simulink model "LunarMicrogrid_Full"  (R2026b)
settings: Solver=ode23t  StopTime=simulation.timeSim  MaxStep=1/(5*solarPlant.converterSwitchingFrequency)  AbsTol=1e-3
PreLoadFcn:
  | run('LunarMicrogridA_Data');
values from neighbouring files (symbols this model uses):
  Csc = Csc_cell/Ns_sc*Np_sc    (= 200)    [LunarDAB_Params.m]
  eta_sc = 0.95    [LunarDAB_Params.m]
  fsw = 100e3    (= 100000)    [LunarDAB_Params.m]
  k_restore = 1    [LunarDAB_Params.m]
  kiCurrent = 2    [LunarDAB_Params.m]
  kiVoltage = 8    [LunarDAB_Params.m]
  kpCurrent = 0.005    [LunarDAB_Params.m]
  kpVoltage = 0.4    [LunarDAB_Params.m]
  lTotal = lSeries + Llk    [LunarDAB_Params.m]
  P170_dt = 1e-4    (= 0.0001)    [P170_PV_Initialize.m]
  P170_Imp = im(ix)    [P170_PV_Initialize.m]
  P170_Vmp = vm(ix)    [P170_PV_Initialize.m]
  Rd_bat = dV_droop/Ibat_max    (= 0.232258064516)    [LunarDAB_Params.m]
  SC_enable = 1    [LunarDAB_Params.m]
  thetaIC = 0    [LunarDAB_Params.m]
  thetaMaxDab = pi/4    (= 0.785398163397)    [LunarDAB_Params.m]
  Tsw = 1/fsw    (= 1e-05)    [LunarDAB_Params.m]
  Vsc0 = sqrt((Vsc_max^2 + Vsc_min^2)/2)    [LunarDAB_Params.m]
  Vsc_max = 119    [LunarDAB_Params.m]
  Vsc_min = 66    [LunarDAB_Params.m]
undefined symbols (not defined in the file or in its folder): a_lpf_sys, battery, bms, connectedLoad, dcVoltage, DiscIntNeverNeededParam, eta_dab, Ibat_sign, mmc, Ndab, P170_T, pvDroop, sc, sensor, socLimit, solarPlant
libraries: sl_discontinuities x13, fl_lib x13, nesl_utility x13, simulink x7, batteryecm_lib x1, simulink_extras x1, ee_lib x1
(part 5 of 8)

== system LunarMicrogrid_Full/BESS Controller/PIctrl/Saturation ==
  In1 : Inport  SampleTime=SampleTime
  Upper Limit : Inport  Port=2  SampleTime=SampleTime
  Lower Limit : Inport  Port=3  SampleTime=SampleTime
  Enabled : Subsystem  VariantControl=Enabled
  External : Subsystem  VariantControl=External
  Passthrough : Subsystem  VariantControl=Disabled
  Out1 : Outport  SampleTime=SampleTime

== system LunarMicrogrid_Full/BESS Controller/PIctrl/Saturation Fdbk ==
  In1 : Inport  SampleTime=SampleTime
  Upper Limit : Inport  Port=2  SampleTime=SampleTime
  Lower Limit : Inport  Port=3  SampleTime=SampleTime
  Disabled : Subsystem  VariantControl=Disabled
  Enabled : Subsystem  VariantControl=Enabled
  External : Subsystem  VariantControl=External
  Passthrough : Subsystem  VariantControl=Passthrough
  Out1 : Outport  SampleTime=SampleTime

== system LunarMicrogrid_Full/BESS Controller/PIctrl/Sum ==
  P : Inport  SampleTime=SampleTime
  I : Inport  Port=2  SampleTime=SampleTime
  D : Inport  Port=3  SampleTime=SampleTime
  Passthrough_I : Subsystem  VariantControl=Passthrough_I
  Passthrough_P : Subsystem  VariantControl=Passthrough_P
  Sum_PD : Subsystem  VariantControl=Sum_PD
  Sum_PI : Subsystem  VariantControl=Sum_PI
  Sum_PID : Subsystem  VariantControl=Sum_PID
  Out1 : Outport  SampleTime=SampleTime

== system LunarMicrogrid_Full/BESS Controller/PIctrl/Sum Fdbk ==
  fromP : Inport  SampleTime=SampleTime
  fromState : Inport  Port=2  SampleTime=SampleTime
  fromD : Inport  Port=3  SampleTime=SampleTime
  Disabled : Subsystem  VariantControl=Disabled
  Enabled : Subsystem  VariantControl=Enabled
  Passthrough : Subsystem  VariantControl=Passthrough
  Out1 : Outport  SampleTime=SampleTime

== system LunarMicrogrid_Full/BESS Controller/PIctrl/Tracking Mode ==
  uout : Inport  SampleTime=SampleTime
  TR : Inport  Port=2  SampleTime=SampleTime
  Disabled : Subsystem  VariantControl=Disabled
  Enabled : Subsystem  VariantControl=Enabled
  Out1 : Outport  SampleTime=SampleTime

== system LunarMicrogrid_Full/BESS Controller/PIctrl/Tracking Mode Sum ==
  fromIgain : Inport  SampleTime=SampleTime
  fromTR : Inport  Port=2  SampleTime=SampleTime
  Passthrough : Subsystem  VariantControl=Passthrough
  Tracking Mode : Subsystem  VariantControl=TrackingMode
  preInt : Outport

== system LunarMicrogrid_Full/BESS Controller/PIctrl/Tsamp - Integral ==
  U : Inport  SampleTime=SampleTime
  Ts : Inport  Port=2  SampleTime=SampleTime
  Disabled : Subsystem  VariantControl=Disabled
  External Ts : Subsystem  VariantControl=ExternalTs
  Passthrough : Subsystem  VariantControl=Passthrough
  TsSignalSpecification : Subsystem  VariantControl=Disabled_SignalSpec
  Out1 : Outport  SampleTime=SampleTime

== system LunarMicrogrid_Full/BESS Controller/PIctrl/Tsamp - Ngain ==
  U : Inport  SampleTime=SampleTime
  Ts : Inport  Port=2  SampleTime=SampleTime
  External Ts : Subsystem  VariantControl=ExternalTs
  Passthrough : Subsystem  VariantControl=Passthrough
  Out1 : Outport  SampleTime=SampleTime

== system LunarMicrogrid_Full/BESS Controller/PIctrl/postSat Signal ==
  feedback : Inport  SampleTime=SampleTime
  forward : Inport  Port=2  SampleTime=SampleTime
  Feedback_Path : Subsystem  VariantControl=Feedback
  Forward_Path : Subsystem  VariantControl=Forward
  Out1 : Outport  SampleTime=SampleTime

== system LunarMicrogrid_Full/BESS Controller/PIctrl/preInt Signal ==
  preInt : Inport  SampleTime=SampleTime
  extAW : Inport  Port=2  SampleTime=SampleTime
  External PreInt : Subsystem  VariantControl=ExternalPreInt
  Internal PreInt : Subsystem  VariantControl=InternalPreInt
  Out1 : Outport  SampleTime=SampleTime

== system LunarMicrogrid_Full/BESS Controller/PIctrl/preSat Signal ==
  feedback : Inport  SampleTime=SampleTime
  forward : Inport  Port=2  SampleTime=SampleTime
  Feedback_Path : Subsystem  VariantControl=Feedback
  Forward_Path : Subsystem  VariantControl=Forward
  Out1 : Outport  SampleTime=SampleTime

== system LunarMicrogrid_Full/PV System Monitoring Panel/Monitoring/Efficiency Calculation ==
  Abs : Abs  SaturateOnIntegerOverflow=off
  Add : Sum
  Add1 : Sum
  Constant : Constant  Value=100e3
  Constant1 : Constant  Value=100e3
  Divide : Product  Inputs=/*
  Divide1 : Product  Inputs=/*
  Gain : Gain  Gain=100
  Switch : Switch  Criteria=u2 > Threshold  SaturateOnIntegerOverflow=off  InputSameDT=off
  Switch1 : Switch  Criteria=u2 > Threshold  SaturateOnIntegerOverflow=off  InputSameDT=off
  Switch2 : Switch  Criteria=u2 > Threshold  SaturateOnIntegerOverflow=off  InputSameDT=off
  Terminator : Terminator
  wires:
  [BatPower] -> Abs/1, Add/2, Switch/2
  [LoadPower] -> Add/1
  [SolarPower] -> Switch1/1, Switch1/2, Add1/2
  Constant/1 -> Switch1/3
  Switch1/1 -> Divide/1
  Add/1 -> Divide/2
  Abs/1 -> Add1/1
  [LoadPower] -> Divide1/2
  Add1/1 -> Switch2/2, Switch2/1
  Constant1/1 -> Switch2/3
  Switch2/1 -> Divide1/1
  Divide/1 -> Switch/1
  Divide1/1 -> Switch/3
  Switch/1 -> Gain/1
  Gain/1 -> Terminator/1  "% Efficiency"

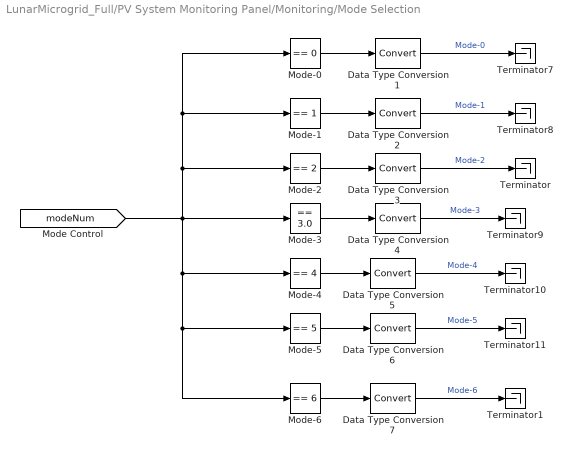
== system LunarMicrogrid_Full/PV System Monitoring Panel/Monitoring/Mode Selection ==
  Data Type Conversion{1..7} (7 alike) : DataTypeConversion  SaturateOnIntegerOverflow=off  RndMeth=Floor
  Mode-0 : simulink/Logic and Bit Operations/Compare To Constant  relop===  const=0  OutDataTypeStr=boolean
  Mode-1 : simulink/Logic and Bit Operations/Compare To Constant  relop===  const=1  OutDataTypeStr=boolean
  Mode-2 : simulink/Logic and Bit Operations/Compare To Constant  relop===  const=2  OutDataTypeStr=boolean
  Mode-3 : simulink/Logic and Bit Operations/Compare To Constant  relop===  const=3.0  OutDataTypeStr=boolean
  Mode-4 : simulink/Logic and Bit Operations/Compare To Constant  relop===  const=4  OutDataTypeStr=boolean
  Mode-5 : simulink/Logic and Bit Operations/Compare To Constant  relop===  const=5  OutDataTypeStr=boolean
  Mode-6 : simulink/Logic and Bit Operations/Compare To Constant  relop===  const=6  OutDataTypeStr=boolean
  Terminator{,1,7..11} (7 alike) : Terminator
  wires:
  Mode-0/1 -> Data Type Conversion1/1
  Mode-3/1 -> Data Type Conversion4/1
  [modeNum] -> Mode-3/1, Mode-4/1, Mode-5/1, Mode-6/1, Mode-2/1, Mode-1/1, Mode-0/1
  Mode-4/1 -> Data Type Conversion5/1
  Mode-1/1 -> Data Type Conversion2/1
  Mode-2/1 -> Data Type Conversion3/1
  Mode-5/1 -> Data Type Conversion6/1
  Mode-6/1 -> Data Type Conversion7/1
  Data Type Conversion1/1 -> Terminator7/1  "Mode-0"
  Data Type Conversion2/1 -> Terminator8/1  "Mode-1"
  Data Type Conversion3/1 -> Terminator/1  "Mode-2"
  Data Type Conversion4/1 -> Terminator9/1  "Mode-3"
  Data Type Conversion5/1 -> Terminator10/1  "Mode-4"
  Data Type Conversion6/1 -> Terminator11/1  "Mode-5"
  Data Type Conversion7/1 -> Terminator1/1  "Mode-6"

== system LunarMicrogrid_Full/BESS Controller/DABCtrl2/Anti-windup/Back Calculation ==
  preSat : Inport  SampleTime=SampleTime
  postSat : Inport  Port=2  SampleTime=SampleTime
  preInt : Inport  Port=3  SampleTime=SampleTime
  P : Inport  Port=4  SampleTime=SampleTime
  Kb : Gain  Gain=Kb  ParamMin=KbParamMin  ParamMax=KbParamMax  OutMin=KbOutMin  OutMax=KbOutMax  RndMeth=Simplest
  Signal Specification2 : SignalSpecification  DisableCoverage=on  OutDataTypeStr=boolean  SampleTime=SampleTime
  SumI2 : Sum  DisableCoverage=on  Inputs=|-+  OutMin=SumI2OutMin  OutMax=SumI2OutMax  RndMeth=Simplest
  SumI4 : Sum  DisableCoverage=on  Inputs=|++  OutMin=SumI4OutMin  OutMax=SumI4OutMax  RndMeth=Simplest
  Terminator2 : Terminator
  Out1 : Outport  SampleTime=SampleTime
  wires:
  preSat/1 -> SumI2/1
  postSat/1 -> SumI2/2
  SumI2/1 -> Kb/1
  Kb/1 -> SumI4/1
  SumI4/1 -> Out1/1
  preInt/1 -> SumI4/2
  Signal Specification2/1 -> Terminator2/1
  P/1 -> Signal Specification2/1

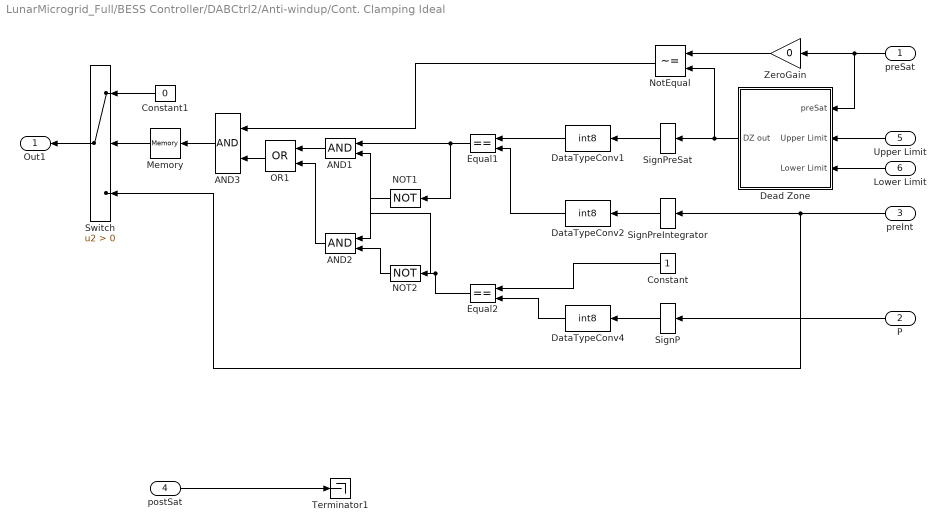
== system LunarMicrogrid_Full/BESS Controller/DABCtrl2/Anti-windup/Cont. Clamping Ideal ==
  preSat : Inport  SampleTime=SampleTime
  P : Inport  Port=2  SampleTime=SampleTime
  preInt : Inport  Port=3  SampleTime=SampleTime
  postSat : Inport  Port=4  SampleTime=SampleTime
  Upper Limit : Inport  Port=5  SampleTime=SampleTime
  Lower Limit : Inport  Port=6  SampleTime=SampleTime
  AND1 : Logic  DisableCoverage=on  OutDataTypeStr=boolean
  AND2 : Logic  DisableCoverage=on  OutDataTypeStr=boolean
  AND3 : Logic  DisableCoverage=on  OutDataTypeStr=boolean
  Constant : Constant  DisableCoverage=on  OutDataTypeStr=int8  PreserveConstantTs=on
  Constant1 : Constant  DisableCoverage=on  Value=0  OutDataTypeStr=Inherit: Inherit via back propagation  PreserveConstantTs=on
  DataTypeConv1 : DataTypeConversion  DisableCoverage=on  OutDataTypeStr=int8  RndMeth=Simplest  SaturateOnIntegerOverflow=off
  DataTypeConv2 : DataTypeConversion  DisableCoverage=on  OutDataTypeStr=int8  RndMeth=Simplest  SaturateOnIntegerOverflow=off
  DataTypeConv4 : DataTypeConversion  DisableCoverage=on  OutDataTypeStr=int8  RndMeth=Simplest  SaturateOnIntegerOverflow=off
  Dead Zone : Subsystem  Variant=on  VariantControlMode=label  LabelModeActiveChoice=External  EmptyChoice=on
  Equal1 : RelationalOperator  DisableCoverage=on  Operator===  OutDataTypeStr=boolean  RndMeth=Simplest  InputSameDT=off
  Equal2 : RelationalOperator  DisableCoverage=on  Operator===  OutDataTypeStr=boolean  RndMeth=Simplest  InputSameDT=off
  Memory : Memory  DisableCoverage=on  InheritSampleTime=on
  NOT1 : Logic  DisableCoverage=on  Operator=NOT  OutDataTypeStr=boolean
  NOT2 : Logic  DisableCoverage=on  Operator=NOT  OutDataTypeStr=boolean
  NotEqual : RelationalOperator  DisableCoverage=on  Operator=~=  OutDataTypeStr=boolean  RndMeth=Simplest  InputSameDT=off
  OR1 : Logic  DisableCoverage=on  Operator=OR  OutDataTypeStr=boolean
  SignP : Signum  DisableCoverage=on
  SignPreIntegrator : Signum  DisableCoverage=on
  SignPreSat : Signum  DisableCoverage=on
  Switch : Switch  Criteria=u2 > Threshold  RndMeth=Simplest  SaturateOnIntegerOverflow=off
  Terminator1 : Terminator
  ZeroGain : Gain  DisableCoverage=on  Gain=0  RndMeth=Simplest  OutDataTypeStr=Inherit: Same as input  ParamDataTypeStr=Inherit: Same as input
  Out1 : Outport  SampleTime=SampleTime
  wires:
  Upper Limit/1 -> Dead Zone/2(Upper Limit)
  Lower Limit/1 -> Dead Zone/3(Lower Limit)
  DataTypeConv4/1 -> Equal2/2
  Constant/1 -> Equal2/1
  DataTypeConv2/1 -> Equal1/2
  DataTypeConv1/1 -> Equal1/1
  AND3/1 -> Memory/1
  OR1/1 -> AND3/2
  AND2/1 -> OR1/2
  AND1/1 -> OR1/1
  NOT2/1 -> AND2/2
  NOT1/1 -> AND2/1
  Equal2/1 -> NOT2/1, AND1/2
  Equal1/1 -> AND1/1, NOT1/1
  NotEqual/1 -> AND3/1
  SignP/1 -> DataTypeConv4/1
  SignPreIntegrator/1 -> DataTypeConv2/1
  SignPreSat/1 -> DataTypeConv1/1
  P/1 -> SignP/1
  preInt/1 -> Switch/3, SignPreIntegrator/1
  Dead Zone/1(DZ out) -> SignPreSat/1, NotEqual/2
  ZeroGain/1 -> NotEqual/1
  preSat/1 -> ZeroGain/1, Dead Zone/1(preSat)
  Switch/1 -> Out1/1
  Constant1/1 -> Switch/1
  Memory/1 -> Switch/2
  postSat/1 -> Terminator1/1

== system LunarMicrogrid_Full/BESS Controller/DABCtrl2/Anti-windup/Cont. Clamping Parallel ==
  preSat : Inport  SampleTime=SampleTime
  preInt : Inport  Port=2  SampleTime=SampleTime
  postSat : Inport  Port=3  SampleTime=SampleTime
  P : Inport  Port=4  SampleTime=SampleTime
  Upper Limit : Inport  Port=5  SampleTime=SampleTime
  Lower Limit : Inport  Port=6  SampleTime=SampleTime
  AND3 : Logic  DisableCoverage=on  OutDataTypeStr=boolean
  Constant1 : Constant  DisableCoverage=on  Value=0  OutDataTypeStr=Inherit: Inherit via back propagation  PreserveConstantTs=on
  DataTypeConv1 : DataTypeConversion  DisableCoverage=on  OutDataTypeStr=int8  RndMeth=Simplest  SaturateOnIntegerOverflow=off
  DataTypeConv2 : DataTypeConversion  DisableCoverage=on  OutDataTypeStr=int8  RndMeth=Simplest  SaturateOnIntegerOverflow=off
  Dead Zone : Subsystem  Variant=on  VariantControlMode=label  LabelModeActiveChoice=External  EmptyChoice=on
  Equal1 : RelationalOperator  DisableCoverage=on  Operator===  OutDataTypeStr=boolean  RndMeth=Simplest  InputSameDT=off
  Memory : Memory  DisableCoverage=on  InheritSampleTime=on
  NotEqual : RelationalOperator  DisableCoverage=on  Operator=~=  OutDataTypeStr=boolean  RndMeth=Simplest  InputSameDT=off
  SignPreIntegrator : Signum  DisableCoverage=on
  SignPreSat : Signum  DisableCoverage=on
  Signal Specification2 : SignalSpecification  DisableCoverage=on  OutDataTypeStr=boolean  SampleTime=SampleTime
  Switch : Switch  Criteria=u2 > Threshold  RndMeth=Simplest  SaturateOnIntegerOverflow=off
  Terminator1 : Terminator
  Terminator2 : Terminator
  ZeroGain : Gain  DisableCoverage=on  Gain=0  RndMeth=Simplest  OutDataTypeStr=Inherit: Same as input  ParamDataTypeStr=Inherit: Same as input
  Out1 : Outport  SampleTime=SampleTime
  wires:
  Upper Limit/1 -> Dead Zone/2(Upper Limit)
  Lower Limit/1 -> Dead Zone/3(Lower Limit)
  AND3/1 -> Memory/1
  Constant1/1 -> Switch/1
  DataTypeConv2/1 -> Equal1/2
  DataTypeConv1/1 -> Equal1/1
  Equal1/1 -> AND3/2
  NotEqual/1 -> AND3/1
  SignPreIntegrator/1 -> DataTypeConv2/1
  SignPreSat/1 -> DataTypeConv1/1
  preInt/1 -> SignPreIntegrator/1, Switch/3
  Dead Zone/1(DZ out) -> SignPreSat/1, NotEqual/2
  ZeroGain/1 -> NotEqual/1
  preSat/1 -> ZeroGain/1, Dead Zone/1(preSat)
  Switch/1 -> Out1/1
  Memory/1 -> Switch/2
  Signal Specification2/1 -> Terminator2/1
  postSat/1 -> Terminator1/1
  P/1 -> Signal Specification2/1

== system LunarMicrogrid_Full/BESS Controller/DABCtrl2/Anti-windup/Disabled ==
  preInt : Inport  SampleTime=SampleTime
  preSat : Inport  Port=2  SampleTime=SampleTime
  postSat : Inport  Port=3  SampleTime=SampleTime
  P : Inport  Port=4  SampleTime=SampleTime
  Signal Specification1 : SignalSpecification  DisableCoverage=on  OutDataTypeStr=boolean  SampleTime=SampleTime
  Signal Specification2 : SignalSpecification  DisableCoverage=on  OutDataTypeStr=boolean  SampleTime=SampleTime
  Terminator{,1..3} (4 alike) : Terminator
  wires:
  postSat/1 -> Terminator1/1
  Signal Specification2/1 -> Terminator2/1
  P/1 -> Signal Specification2/1
  preSat/1 -> Terminator/1
  preInt/1 -> Signal Specification1/1
  Signal Specification1/1 -> Terminator3/1

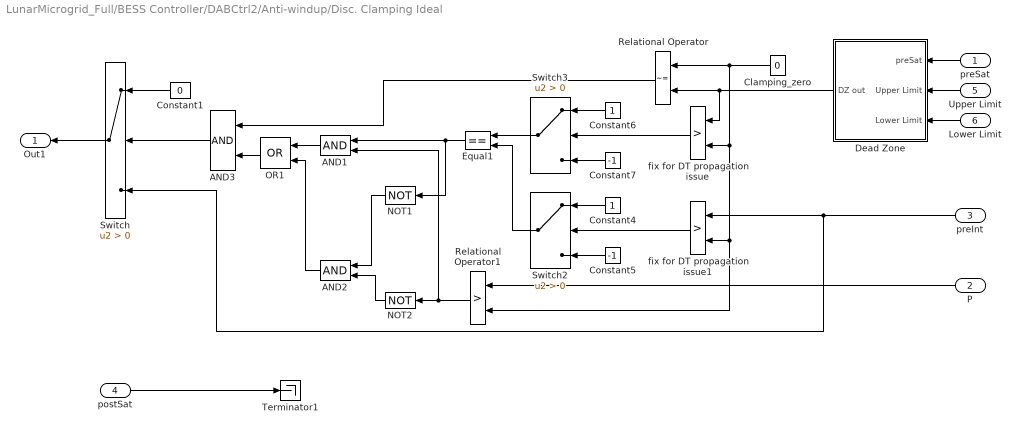
== system LunarMicrogrid_Full/BESS Controller/DABCtrl2/Anti-windup/Disc. Clamping Ideal ==
  preSat : Inport  SampleTime=SampleTime
  P : Inport  Port=2  SampleTime=SampleTime
  preInt : Inport  Port=3  SampleTime=SampleTime
  postSat : Inport  Port=4  SampleTime=SampleTime
  Upper Limit : Inport  Port=5  SampleTime=SampleTime
  Lower Limit : Inport  Port=6  SampleTime=SampleTime
  AND1 : Logic  DisableCoverage=on  OutDataTypeStr=boolean
  AND2 : Logic  DisableCoverage=on  OutDataTypeStr=boolean
  AND3 : Logic  DisableCoverage=on  OutDataTypeStr=boolean
  Clamping_zero : Constant  DisableCoverage=on  Value=0  OutMin=ClampingZeroOutMin  OutMax=ClampingZeroOutMax  OutDataTypeStr=Inherit: Inherit via back propagation
  Constant1 : Constant  DisableCoverage=on  Value=0  OutDataTypeStr=Inherit: Inherit via back propagation  PreserveConstantTs=on
  Constant4 : Constant  DisableCoverage=on  OutDataTypeStr=int8
  Constant5 : Constant  DisableCoverage=on  Value=-1  OutDataTypeStr=int8
  Constant6 : Constant  DisableCoverage=on  OutDataTypeStr=int8
  Constant7 : Constant  DisableCoverage=on  Value=-1  OutDataTypeStr=int8
  Dead Zone : Subsystem  Variant=on  VariantControlMode=label  LabelModeActiveChoice=External  EmptyChoice=on
  Equal1 : RelationalOperator  DisableCoverage=on  Operator===  OutDataTypeStr=boolean  RndMeth=Simplest  InputSameDT=off
  NOT1 : Logic  DisableCoverage=on  Operator=NOT  OutDataTypeStr=boolean
  NOT2 : Logic  DisableCoverage=on  Operator=NOT  OutDataTypeStr=boolean
  OR1 : Logic  DisableCoverage=on  Operator=OR  OutDataTypeStr=boolean
  Relational Operator : RelationalOperator  DisableCoverage=on  Operator=~=  OutDataTypeStr=boolean  RndMeth=Simplest  InputSameDT=off
  Relational Operator1 : RelationalOperator  DisableCoverage=on  Operator=>  OutDataTypeStr=boolean  RndMeth=Simplest  InputSameDT=off
  Switch : Switch  Criteria=u2 > Threshold  RndMeth=Simplest  SaturateOnIntegerOverflow=off
  Switch2 : Switch  DisableCoverage=on  Criteria=u2 > Threshold  SaturateOnIntegerOverflow=off  InputSameDT=off
  Switch3 : Switch  DisableCoverage=on  Criteria=u2 > Threshold  SaturateOnIntegerOverflow=off  InputSameDT=off
  Terminator1 : Terminator
  fix for DT propagation issue : RelationalOperator  DisableCoverage=on  Operator=>  OutDataTypeStr=boolean  RndMeth=Simplest  InputSameDT=off
  fix for DT propagation issue1 : RelationalOperator  DisableCoverage=on  Operator=>  OutDataTypeStr=boolean  RndMeth=Simplest  InputSameDT=off
  Out1 : Outport  SampleTime=SampleTime
  wires:
  fix for DT propagation issue1/1 -> Switch2/2
  P/1 -> Relational Operator1/1
  Relational Operator/1 -> AND3/1
  Dead Zone/1(DZ out) -> Relational Operator/2, fix for DT propagation issue/1
  fix for DT propagation issue/1 -> Switch3/2
  Clamping_zero/1 -> fix for DT propagation issue/2, fix for DT propagation issue1/2, Relational Operator1/2, Relational Operator/1
  Switch2/1 -> Equal1/2
  Switch3/1 -> Equal1/1
  Constant7/1 -> Switch3/3
  Constant6/1 -> Switch3/1
  Constant4/1 -> Switch2/1
  Constant5/1 -> Switch2/3
  Lower Limit/1 -> Dead Zone/3(Lower Limit)
  Upper Limit/1 -> Dead Zone/2(Upper Limit)
  Switch/1 -> Out1/1
  AND3/1 -> Switch/2
  Constant1/1 -> Switch/1
  OR1/1 -> AND3/2
  AND2/1 -> OR1/2
  AND1/1 -> OR1/1
  NOT2/1 -> AND2/2
  NOT1/1 -> AND2/1
  Relational Operator1/1 -> NOT2/1, AND1/2
  Equal1/1 -> AND1/1, NOT1/1
  preInt/1 -> fix for DT propagation issue1/1, Switch/3
  preSat/1 -> Dead Zone/1(preSat)
  postSat/1 -> Terminator1/1

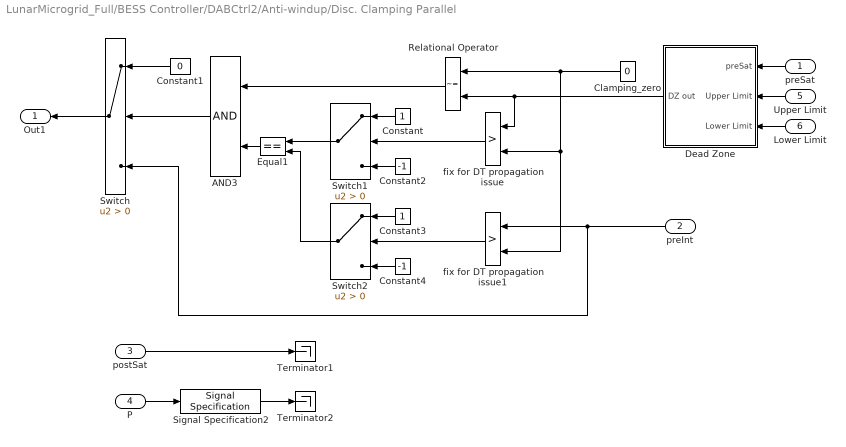
== system LunarMicrogrid_Full/BESS Controller/DABCtrl2/Anti-windup/Disc. Clamping Parallel ==
  preSat : Inport  SampleTime=SampleTime
  preInt : Inport  Port=2  SampleTime=SampleTime
  postSat : Inport  Port=3  SampleTime=SampleTime
  P : Inport  Port=4  SampleTime=SampleTime
  Upper Limit : Inport  Port=5  SampleTime=SampleTime
  Lower Limit : Inport  Port=6  SampleTime=SampleTime
  AND3 : Logic  DisableCoverage=on  OutDataTypeStr=boolean
  Clamping_zero : Constant  DisableCoverage=on  Value=0  OutMin=ClampingZeroOutMin  OutMax=ClampingZeroOutMax  OutDataTypeStr=Inherit: Inherit via back propagation
  Constant : Constant  DisableCoverage=on  OutDataTypeStr=int8
  Constant1 : Constant  DisableCoverage=on  Value=0  OutDataTypeStr=Inherit: Inherit via back propagation  PreserveConstantTs=on
  Constant2 : Constant  DisableCoverage=on  Value=-1  OutDataTypeStr=int8
  Constant3 : Constant  DisableCoverage=on  OutDataTypeStr=int8
  Constant4 : Constant  DisableCoverage=on  Value=-1  OutDataTypeStr=int8
  Dead Zone : Subsystem  Variant=on  VariantControlMode=label  LabelModeActiveChoice=External  EmptyChoice=on
  Equal1 : RelationalOperator  DisableCoverage=on  Operator===  OutDataTypeStr=boolean  RndMeth=Simplest  InputSameDT=off
  Relational Operator : RelationalOperator  DisableCoverage=on  Operator=~=  OutDataTypeStr=boolean  RndMeth=Simplest  InputSameDT=off
  Signal Specification2 : SignalSpecification  DisableCoverage=on  OutDataTypeStr=boolean  SampleTime=SampleTime
  Switch : Switch  Criteria=u2 > Threshold  RndMeth=Simplest  SampleTime=SampleTime  SaturateOnIntegerOverflow=off
  Switch1 : Switch  DisableCoverage=on  Criteria=u2 > Threshold  SaturateOnIntegerOverflow=off  InputSameDT=off
  Switch2 : Switch  DisableCoverage=on  Criteria=u2 > Threshold  SaturateOnIntegerOverflow=off  InputSameDT=off
  Terminator1 : Terminator
  Terminator2 : Terminator
  fix for DT propagation issue : RelationalOperator  DisableCoverage=on  Operator=>  OutDataTypeStr=boolean  RndMeth=Simplest  InputSameDT=off
  fix for DT propagation issue1 : RelationalOperator  DisableCoverage=on  Operator=>  OutDataTypeStr=boolean  RndMeth=Simplest  InputSameDT=off
  Out1 : Outport  SampleTime=SampleTime
  wires:
  fix for DT propagation issue1/1 -> Switch2/2
  fix for DT propagation issue/1 -> Switch1/2
  Clamping_zero/1 -> fix for DT propagation issue/2, fix for DT propagation issue1/2, Relational Operator/1
  Constant1/1 -> Switch/1
  Switch2/1 -> Equal1/2
  Constant3/1 -> Switch2/1
  Constant4/1 -> Switch2/3
  Switch1/1 -> Equal1/1
  preInt/1 -> Switch/3, fix for DT propagation issue1/1
  Constant2/1 -> Switch1/3
  Constant/1 -> Switch1/1
  Relational Operator/1 -> AND3/1
  Lower Limit/1 -> Dead Zone/3(Lower Limit)
  Upper Limit/1 -> Dead Zone/2(Upper Limit)
  preSat/1 -> Dead Zone/1(preSat)
  Dead Zone/1(DZ out) -> Relational Operator/2, fix for DT propagation issue/1
  Equal1/1 -> AND3/2
  AND3/1 -> Switch/2
  Switch/1 -> Out1/1
  Signal Specification2/1 -> Terminator2/1
  postSat/1 -> Terminator1/1
  P/1 -> Signal Specification2/1

== system LunarMicrogrid_Full/BESS Controller/DABCtrl2/Anti-windup/Passthrough ==
  preInt : Inport  SampleTime=SampleTime
  preSat : Inport  Port=2  SampleTime=SampleTime
  postSat : Inport  Port=3  SampleTime=SampleTime
  P : Inport  Port=4  SampleTime=SampleTime
  Signal Specification2 : SignalSpecification  DisableCoverage=on  OutDataTypeStr=boolean  SampleTime=SampleTime
  Terminator : Terminator
  Terminator1 : Terminator
  Terminator2 : Terminator
  Out1 : Outport  SampleTime=SampleTime
  wires:
  preInt/1 -> Out1/1
  preSat/1 -> Terminator/1
  postSat/1 -> Terminator1/1
  P/1 -> Signal Specification2/1
  Signal Specification2/1 -> Terminator2/1

== system LunarMicrogrid_Full/BESS Controller/DABCtrl2/D Gain/Disabled ==
  D Gain : Inport  SampleTime=SampleTime
  Signal Specification : SignalSpecification  DisableCoverage=on  OutDataTypeStr=boolean  SampleTime=SampleTime
  Terminator : Terminator
  wires:
  D Gain/1 -> Signal Specification/1
  Signal Specification/1 -> Terminator/1

== system LunarMicrogrid_Full/BESS Controller/DABCtrl2/D Gain/External Parameters ==
  err : Inport  SampleTime=SampleTime
  D Gain : Inport  Port=2  SampleTime=SampleTime
  DProd Out : Product  OutMin=DOutMin  OutMax=DOutMax  RndMeth=Simplest  SampleTime=SampleTime
  Out1 : Outport  SampleTime=SampleTime
  wires:
  DProd Out/1 -> Out1/1
  D Gain/1 -> DProd Out/2
  err/1 -> DProd Out/1

== system LunarMicrogrid_Full/BESS Controller/DABCtrl2/D Gain/Internal Parameters ==
  err : Inport  SampleTime=SampleTime
  D Gain : Inport  Port=2  SampleTime=SampleTime
  Derivative Gain : Gain  DisableCoverage=on  Gain=D  ParamMin=DParamMin  ParamMax=DParamMax  OutMin=DOutMin  OutMax=DOutMax  RndMeth=Simplest
  Signal Specification : SignalSpecification  DisableCoverage=on  OutDataTypeStr=boolean  SampleTime=SampleTime
  Terminator : Terminator
  Out1 : Outport  SampleTime=SampleTime
  wires:
  Derivative Gain/1 -> Out1/1
  err/1 -> Derivative Gain/1
  D Gain/1 -> Signal Specification/1
  Signal Specification/1 -> Terminator/1

== system LunarMicrogrid_Full/BESS Controller/DABCtrl2/External Derivative/Disabled ==
  ydot : Inport  SampleTime=SampleTime
  err : Inport  Port=2  SampleTime=SampleTime
  Signal Specification : SignalSpecification  DisableCoverage=on  OutDataTypeStr=boolean  SampleTime=SampleTime
  Terminator1 : Terminator
  Out1 : Outport  SampleTime=SampleTime
  wires:
  err/1 -> Terminator1/1
  Signal Specification/1 -> Out1/1
  ydot/1 -> Signal Specification/1

== system LunarMicrogrid_Full/BESS Controller/DABCtrl2/External Derivative/Error ==
  err : Inport  SampleTime=SampleTime
  ydot : Inport  Port=2  SampleTime=SampleTime
  Signal Specification : SignalSpecification  DisableCoverage=on  OutDataTypeStr=boolean  SampleTime=SampleTime
  Terminator : Terminator
  Out1 : Outport  SampleTime=SampleTime
  wires:
  Signal Specification/1 -> Terminator/1
  ydot/1 -> Signal Specification/1
  err/1 -> Out1/1

== system LunarMicrogrid_Full/BESS Controller/DABCtrl2/External Derivative/External Ydot ==
  err : Inport  SampleTime=SampleTime
  ydot : Inport  Port=2  SampleTime=SampleTime
  Terminator : Terminator
  Unary Minus : UnaryMinus
  Out1 : Outport  SampleTime=SampleTime
  wires:
  Unary Minus/1 -> Out1/1
  err/1 -> Terminator/1
  ydot/1 -> Unary Minus/1

== system LunarMicrogrid_Full/BESS Controller/DABCtrl2/Filter/Cont. Filter ==
  U : Inport  SampleTime=SampleTime
  Nout : Inport  Port=2  SampleTime=SampleTime
  Reset : Inport  Port=3  SampleTime=SampleTime
  D0in : Inport  Port=4  SampleTime=SampleTime
  N : Inport  Port=5  SampleTime=SampleTime
  Ts : Inport  Port=6  SampleTime=SampleTime
  Filter : Integrator  DisableCoverage=on
  Signal Specification2 : SignalSpecification  DisableCoverage=on  OutDataTypeStr=boolean  SampleTime=SampleTime
  SumD : Sum  DisableCoverage=on  Inputs=|+-  OutMin=SumDOutMin  OutMax=SumDOutMax  RndMeth=Simplest
  Terminator{,1..3} (4 alike) : Terminator
  Y : Outport  SampleTime=SampleTime
  wires:
  Ts/1 -> Terminator3/1
  D0in/1 -> Terminator/1
  U/1 -> SumD/1
  Filter/1 -> SumD/2
  SumD/1 -> Y/1
  Nout/1 -> Filter/1
  N/1 -> Signal Specification2/1
  Signal Specification2/1 -> Terminator2/1
  Reset/1 -> Terminator1/1

== system LunarMicrogrid_Full/BESS Controller/DABCtrl2/Filter/Cont. Filter Only ==
  U : Inport  SampleTime=SampleTime
  Nout : Inport  Port=2  SampleTime=SampleTime
  Reset : Inport  Port=3  SampleTime=SampleTime
  D0in : Inport  Port=4  SampleTime=SampleTime
  N : Inport  Port=5  SampleTime=SampleTime
  Ts : Inport  Port=6  SampleTime=SampleTime
  Filter : Integrator  DisableCoverage=on  InitialCondition=InitialConditionForFilter
  Signal Specification2 : SignalSpecification  DisableCoverage=on  OutDataTypeStr=boolean  SampleTime=SampleTime
  SumD : Sum  DisableCoverage=on  Inputs=|+-  OutMin=SumDOutMin  OutMax=SumDOutMax
  Terminator{,1..3} (4 alike) : Terminator
  Y : Outport  SampleTime=SampleTime
  wires:
  Nout/1 -> SumD/2
  Filter/1 -> Y/1
  SumD/1 -> Filter/1
  Ts/1 -> Terminator3/1
  D0in/1 -> Terminator/1
  U/1 -> SumD/1
  N/1 -> Signal Specification2/1
  Signal Specification2/1 -> Terminator2/1
  Reset/1 -> Terminator1/1

== system LunarMicrogrid_Full/BESS Controller/DABCtrl2/Filter/Differentiator ==
  U : Inport  SampleTime=SampleTime
  Reset : Inport  Port=2  SampleTime=SampleTime
  D0in : Inport  Port=3  SampleTime=SampleTime
  Nout : Inport  Port=4  SampleTime=SampleTime
  N : Inport  Port=5  SampleTime=SampleTime
  Ts : Inport  Port=6  SampleTime=SampleTime
  DTDup : DataTypeDuplicate  NumInputPorts=3
  Diff : Sum  Inputs=+-  OutMin=DifferentiatorOutMin  OutMax=DifferentiatorOutMax  OutDataTypeStr=Inherit: Inherit via back propagation  InputSameDT=on  RndMeth=Simplest
  Signal Specification1 : SignalSpecification  DisableCoverage=on  OutDataTypeStr=boolean  SampleTime=SampleTime
  Terminator{,1..3} (4 alike) : Terminator
  Tsamp : Subsystem  Variant=on  VariantControlMode=label  LabelModeActiveChoice=InternalTs
  UD : Delay  DelayLength=1  InitialCondition=DifferentiatorICPrevScaledInput  SampleTime=SampleTime
  Y : Outport  OutMin=DifferentiatorOutMin  OutMax=DifferentiatorOutMax  SampleTime=SampleTime
  wires:
  Ts/1 -> Tsamp/2(Ts)
  D0in/1 -> Terminator/1
  U/1 -> Tsamp/1(U)
  UD/1 -> Diff/2, DTDup/3
  Tsamp/1(Out1) -> Diff/1, UD/1, DTDup/2
  Diff/1 -> Y/1, DTDup/1
  Nout/1 -> Terminator2/1
  N/1 -> Signal Specification1/1
  Signal Specification1/1 -> Terminator1/1
  Reset/1 -> Terminator3/1

== system LunarMicrogrid_Full/BESS Controller/DABCtrl2/Filter/Disabled ==
  Reset : Inport  SampleTime=SampleTime
  U : Inport  Port=2  SampleTime=SampleTime
  N : Inport  Port=3  SampleTime=SampleTime
  D0in : Inport  Port=4  SampleTime=SampleTime
  Nout : Inport  Port=5  SampleTime=SampleTime
  Ts : Inport  Port=6  SampleTime=SampleTime
  Signal Specification{1..4} (4 alike) : SignalSpecification  DisableCoverage=on  OutDataTypeStr=boolean  SampleTime=SampleTime
  Terminator{1..6} (6 alike) : Terminator
  wires:
  Ts/1 -> Terminator6/1
  U/1 -> Signal Specification3/1
  Signal Specification3/1 -> Terminator3/1
  Signal Specification1/1 -> Terminator1/1
  N/1 -> Signal Specification1/1
  Nout/1 -> Signal Specification2/1
  Signal Specification4/1 -> Terminator4/1
  D0in/1 -> Signal Specification4/1
  Reset/1 -> Terminator5/1
  Signal Specification2/1 -> Terminator2/1

== system LunarMicrogrid_Full/BESS Controller/DABCtrl2/Filter/Disc. Backward Euler Filter ==
  note: Denominator Coefficients
  U : Inport  SampleTime=SampleTime
  N : Inport  Port=2  SampleTime=SampleTime
  Reset : Inport  Port=3  SampleTime=SampleTime
  D0in : Inport  Port=4  SampleTime=SampleTime
  Nout : Inport  Port=5  SampleTime=SampleTime
  Ts : Inport  Port=6  SampleTime=SampleTime
  DenCoefOut : Product  OutMin=FilterDiffOutCoefMin  OutMax=FilterDiffOutCoefMax  RndMeth=Simplest  SampleTime=SampleTime
  Filter Den Constant : Constant  DisableCoverage=on  OutMin=FilterDenConstantOutMin  OutMax=FilterDenConstantOutMax  OutDataTypeStr=Inherit: Inherit via back propagation  PreserveConstantTs=on
  Filter Differentiator TF : DiscreteTransferFcn  Numerator=[1 -1]  DenominatorSource=Input port  SampleTime=SampleTime  a0EqualsOne=on  RndMeth=Simplest
      settings: InputPortMap=u0,p3
  Mux : Mux  Inputs=2
  Passthrough for tuning : DataTypeConversion  Tag=#GainSurfaceTarget_  RndMeth=Simplest  SaturateOnIntegerOverflow=off
  Reciprocal : Math  Operator=reciprocal  OutMin=ReciprocalOutMin  OutMax=ReciprocalOutMax  RndMeth=Simplest  SaturateOnIntegerOverflow=off  OutDataTypeStr=Inherit: Inherit via internal rule
  SumDen : Sum  Inputs=++|  OutMin=SumDenOutMin  OutMax=SumDenOutMax  InputSameDT=on  RndMeth=Simplest
  Terminator : Terminator
  Terminator1 : Terminator
  Terminator2 : Terminator
  Tsamp : Subsystem  Variant=on  VariantControlMode=label  LabelModeActiveChoice=InternalTs
  Unary Minus : UnaryMinus
  Y : Outport  SampleTime=SampleTime
  wires:
  Ts/1 -> Tsamp/2(Ts)
  D0in/1 -> Terminator/1
  Filter Differentiator TF/1 -> DenCoefOut/1
  DenCoefOut/1 -> Y/1
  U/1 -> Filter Differentiator TF/1
  Passthrough for tuning/1 -> Tsamp/1(N)
  N/1 -> Passthrough for tuning/1
  Filter Den Constant/1 -> SumDen/1, Mux/1
  Tsamp/1(Out1) -> SumDen/2
  Reciprocal/1 -> DenCoefOut/2, Unary Minus/1
  SumDen/1 -> Reciprocal/1
  Unary Minus/1 -> Mux/2
  Mux/1 -> Filter Differentiator TF/2
  Nout/1 -> Terminator2/1
  Reset/1 -> Terminator1/1

== system LunarMicrogrid_Full/BESS Controller/DABCtrl2/Filter/Disc. Backward Euler Filter Only ==
  note: Denominator Coefficients
  U : Inport  SampleTime=SampleTime
  N : Inport  Port=2  SampleTime=SampleTime
  Reset : Inport  Port=3  SampleTime=SampleTime
  D0in : Inport  Port=4  SampleTime=SampleTime
  Nout : Inport  Port=5  SampleTime=SampleTime
  Ts : Inport  Port=6  SampleTime=SampleTime
  DenCoefOut : Product  OutMin=FilterDiffOutCoefMin  OutMax=FilterDiffOutCoefMax  SampleTime=SampleTime
  Filter Den Constant : Constant  DisableCoverage=on  OutMin=FilterDenConstantOutMin  OutMax=FilterDenConstantOutMax  OutDataTypeStr=Inherit: Inherit via back propagation  PreserveConstantTs=on
  Filter Differentiator TF : DiscreteTransferFcn  DenominatorSource=Input port  InitialStates=InitialConditionForFilter  SampleTime=SampleTime  a0EqualsOne=on
      settings: InputPortMap=u0,p3
  Mux : Mux  Inputs=2
  Passthrough for tuning : DataTypeConversion  Tag=#GainSurfaceTarget_  SaturateOnIntegerOverflow=off  RndMeth=Floor
  SumDen : Sum  Inputs=|++  OutMin=SumDenOutMin  OutMax=SumDenOutMax  InputSameDT=on
  Terminator : Terminator
  Terminator1 : Terminator
  Terminator2 : Terminator
  Tsamp : Subsystem  Variant=on  VariantControlMode=label  LabelModeActiveChoice=InternalTs
  Unary Minus : UnaryMinus
  Y : Outport  SampleTime=SampleTime
  wires:
  Filter Den Constant/1 -> Unary Minus/1, SumDen/2
  SumDen/1 -> Mux/1
  Unary Minus/1 -> Mux/2
  Reset/1 -> Terminator1/1
  Nout/1 -> Terminator2/1
  Mux/1 -> Filter Differentiator TF/2
  Tsamp/1(Out1) -> DenCoefOut/2, SumDen/1
  N/1 -> Passthrough for tuning/1
  Passthrough for tuning/1 -> Tsamp/1(N)
  U/1 -> Filter Differentiator TF/1
  DenCoefOut/1 -> Y/1
  Filter Differentiator TF/1 -> DenCoefOut/1
  D0in/1 -> Terminator/1
  Ts/1 -> Tsamp/2(Ts)

== system LunarMicrogrid_Full/BESS Controller/DABCtrl2/Filter/Disc. Forward Euler Filter ==
  U : Inport  SampleTime=SampleTime
  Nout : Inport  Port=2  SampleTime=SampleTime
  Reset : Inport  Port=3  SampleTime=SampleTime
  D0in : Inport  Port=4  SampleTime=SampleTime
  N : Inport  Port=5  SampleTime=SampleTime
  Ts : Inport  Port=6  SampleTime=SampleTime
  Filter : DiscreteIntegrator  DisableCoverage=on  SampleTime=SampleTime  OutMin=FilterOutMin  OutMax=FilterOutMax  RndMeth=Simplest  ICPrevOutput=DiscIntNeverNeededParam  ICPrevScaledInput=DiscIntNeverNeededParam
  Signal Specification2 : SignalSpecification  DisableCoverage=on  OutDataTypeStr=boolean  SampleTime=SampleTime
  SumD : Sum  DisableCoverage=on  Inputs=|+-  OutMin=SumDOutMin  OutMax=SumDOutMax  RndMeth=Simplest
  Terminator{,1..3} (4 alike) : Terminator
  Y : Outport  SampleTime=SampleTime
  wires:
  Ts/1 -> Terminator3/1
  D0in/1 -> Terminator/1
  SumD/1 -> Y/1
  Nout/1 -> Filter/1
  U/1 -> SumD/1
  Filter/1 -> SumD/2
  N/1 -> Signal Specification2/1
  Signal Specification2/1 -> Terminator2/1
  Reset/1 -> Terminator1/1

== system LunarMicrogrid_Full/BESS Controller/DABCtrl2/Filter/Disc. Forward Euler Filter Only ==
  U : Inport  SampleTime=SampleTime
  Nout : Inport  Port=2  SampleTime=SampleTime
  Reset : Inport  Port=3  SampleTime=SampleTime
  D0in : Inport  Port=4  SampleTime=SampleTime
  N : Inport  Port=5  SampleTime=SampleTime
  Ts : Inport  Port=6  SampleTime=SampleTime
  Filter : DiscreteIntegrator  DisableCoverage=on  InitialCondition=InitialConditionForFilter  SampleTime=SampleTime  OutMin=FilterOutMin  OutMax=FilterOutMax  ICPrevOutput=DiscIntNeverNeededParam  ICPrevScaledInput=DiscIntNeverNeededParam
  Signal Specification2 : SignalSpecification  DisableCoverage=on  OutDataTypeStr=boolean  SampleTime=SampleTime
  SumD : Sum  DisableCoverage=on  Inputs=|+-  OutMin=SumDOutMin  OutMax=SumDOutMax
  Terminator{,1..3} (4 alike) : Terminator
  Y : Outport  SampleTime=SampleTime
  wires:
  Filter/1 -> Y/1
  Reset/1 -> Terminator1/1
  Signal Specification2/1 -> Terminator2/1
  N/1 -> Signal Specification2/1
  Nout/1 -> SumD/2
  U/1 -> SumD/1
  SumD/1 -> Filter/1
  D0in/1 -> Terminator/1
  Ts/1 -> Terminator3/1

== system LunarMicrogrid_Full/BESS Controller/DABCtrl2/Filter/Disc. Trapezoidal Filter ==
  note: Denominator Coefficients
  U : Inport  SampleTime=SampleTime
  N : Inport  Port=2  SampleTime=SampleTime
  Reset : Inport  Port=3  SampleTime=SampleTime
  D0in : Inport  Port=4  SampleTime=SampleTime
  Nout : Inport  Port=5  SampleTime=SampleTime
  Ts : Inport  Port=6  SampleTime=SampleTime
  DenCoefOut : Product  OutMin=FilterDiffOutCoefMin  OutMax=FilterDiffOutCoefMax  RndMeth=Simplest  SampleTime=SampleTime
  Divide : Product  InputSameDT=on  OutMin=DivideOutMin  OutMax=DivideOutMax  RndMeth=Simplest  SampleTime=SampleTime
  Filter Den Constant : Constant  DisableCoverage=on  OutMin=FilterDenConstantOutMin  OutMax=FilterDenConstantOutMax  OutDataTypeStr=Inherit: Inherit via back propagation  PreserveConstantTs=on
  Filter Differentiator TF : DiscreteTransferFcn  Numerator=[1 -1]  DenominatorSource=Input port  SampleTime=SampleTime  a0EqualsOne=on  RndMeth=Simplest
      settings: InputPortMap=u0,p3
  Mux : Mux  Inputs=2
  Passthrough for tuning : DataTypeConversion  Tag=#GainSurfaceTarget_  RndMeth=Simplest  SaturateOnIntegerOverflow=off
  Reciprocal : Math  Operator=reciprocal  OutMin=ReciprocalOutMin  OutMax=ReciprocalOutMax  RndMeth=Simplest  SaturateOnIntegerOverflow=off  OutDataTypeStr=Inherit: Inherit via internal rule
  SumDen : Sum  Inputs=++|  OutMin=SumDenOutMin  OutMax=SumDenOutMax  InputSameDT=on  RndMeth=Simplest
  SumNum : Sum  Inputs=-+|  OutMin=SumNumOutMin  OutMax=SumNumOutMax  InputSameDT=on  RndMeth=Simplest
  Terminator : Terminator
  Terminator1 : Terminator
  Terminator2 : Terminator
  Tsamp : Subsystem  Variant=on  VariantControlMode=label  LabelModeActiveChoice=InternalTs
  Y : Outport  SampleTime=SampleTime
  wires:
  Ts/1 -> Tsamp/2(Ts)
  D0in/1 -> Terminator/1
  Passthrough for tuning/1 -> Tsamp/1(N)
  Tsamp/1(Out1) -> SumDen/2, SumNum/2
  Filter Den Constant/1 -> SumNum/1, Mux/1, SumDen/1
  SumDen/1 -> Reciprocal/1
  SumNum/1 -> Divide/2
  Divide/1 -> Mux/2
  Reciprocal/1 -> DenCoefOut/2, Divide/1
  U/1 -> Filter Differentiator TF/1
  Filter Differentiator TF/1 -> DenCoefOut/1
  Mux/1 -> Filter Differentiator TF/2
  N/1 -> Passthrough for tuning/1
  DenCoefOut/1 -> Y/1
  Nout/1 -> Terminator2/1
  Reset/1 -> Terminator1/1

== system LunarMicrogrid_Full/BESS Controller/DABCtrl2/Filter/Disc. Trapezoidal Filter Only ==
  note: Denominator Coefficients
  U : Inport  SampleTime=SampleTime
  N : Inport  Port=2  SampleTime=SampleTime
  Reset : Inport  Port=3  SampleTime=SampleTime
  D0in : Inport  Port=4  SampleTime=SampleTime
  Nout : Inport  Port=5  SampleTime=SampleTime
  Ts : Inport  Port=6  SampleTime=SampleTime
  DenCoefOut : Product  OutMin=FilterDiffOutCoefMin  OutMax=FilterDiffOutCoefMax  SampleTime=SampleTime
  Filter Den Constant : Constant  DisableCoverage=on  Value=2  OutMin=FilterDenConstantOutMin  OutMax=FilterDenConstantOutMax  OutDataTypeStr=Inherit: Inherit via back propagation  PreserveConstantTs=on
  Filter Differentiator TF : DiscreteTransferFcn  Numerator=[1 1]  DenominatorSource=Input port  InitialStates=InitialConditionForFilter  SampleTime=SampleTime  a0EqualsOne=on
      settings: InputPortMap=u0,p3
  Mux : Mux  Inputs=2
  Passthrough for tuning : DataTypeConversion  Tag=#GainSurfaceTarget_  SaturateOnIntegerOverflow=off  RndMeth=Floor
  SumDen : Sum  Inputs=|++  OutMin=SumDenOutMin  OutMax=SumDenOutMax  InputSameDT=on
  SumNum : Sum  Inputs=-+|  OutMin=SumNumOutMin  OutMax=SumNumOutMax  InputSameDT=on
  Terminator : Terminator
  Terminator1 : Terminator
  Terminator2 : Terminator
  Tsamp : Subsystem  Variant=on  VariantControlMode=label  LabelModeActiveChoice=InternalTs
  Y : Outport  SampleTime=SampleTime
  wires:
  SumNum/1 -> Mux/2
  SumDen/1 -> Mux/1
  Filter Den Constant/1 -> SumDen/1, SumNum/1
  Tsamp/1(Out1) -> SumDen/2, SumNum/2, DenCoefOut/2
  Reset/1 -> Terminator1/1
  Nout/1 -> Terminator2/1
  DenCoefOut/1 -> Y/1
  N/1 -> Passthrough for tuning/1
  Mux/1 -> Filter Differentiator TF/2
  Filter Differentiator TF/1 -> DenCoefOut/1
  U/1 -> Filter Differentiator TF/1
  Passthrough for tuning/1 -> Tsamp/1(N)
  D0in/1 -> Terminator/1
  Ts/1 -> Tsamp/2(Ts)

== system LunarMicrogrid_Full/BESS Controller/DABCtrl2/Filter/Passthrough ==
  Reset : Inport  SampleTime=SampleTime
  U : Inport  Port=2  SampleTime=SampleTime
  N : Inport  Port=3  SampleTime=SampleTime
  D0in : Inport  Port=4  SampleTime=SampleTime
  Nout : Inport  Port=5  SampleTime=SampleTime
  Ts : Inport  Port=6  SampleTime=SampleTime
  Signal Specification1 : SignalSpecification  DisableCoverage=on  OutDataTypeStr=boolean  SampleTime=SampleTime
  Signal Specification4 : SignalSpecification  DisableCoverage=on  OutDataTypeStr=boolean  SampleTime=SampleTime
  Terminator{1..2,4..6} (5 alike) : Terminator
  Y : Outport  SampleTime=SampleTime
  wires:
  Nout/1 -> Terminator2/1
  Reset/1 -> Terminator5/1
  D0in/1 -> Signal Specification4/1
  Signal Specification4/1 -> Terminator4/1
  N/1 -> Signal Specification1/1
  Signal Specification1/1 -> Terminator1/1
  U/1 -> Y/1
  Ts/1 -> Terminator6/1

== system LunarMicrogrid_Full/BESS Controller/DABCtrl2/Filter ICs/Disabled ==
  D0 : Inport  SampleTime=SampleTime
  Ground : Ground  DisableCoverage=on
  Signal Specification : SignalSpecification  DisableCoverage=on  OutDataTypeStr=boolean  SampleTime=SampleTime
  Signal Specification1 : SignalSpecification  DisableCoverage=on  OutDataTypeStr=boolean  SampleTime=SampleTime
  Terminator : Terminator
  Out1 : Outport  SampleTime=SampleTime
  wires:
  D0/1 -> Signal Specification/1
  Signal Specification/1 -> Terminator/1
  Ground/1 -> Signal Specification1/1
  Signal Specification1/1 -> Out1/1

== system LunarMicrogrid_Full/BESS Controller/DABCtrl2/Filter ICs/External IC ==
  D0 : Inport  SampleTime=SampleTime
  Out1 : Outport  SampleTime=SampleTime
  wires:
  D0/1 -> Out1/1

== system LunarMicrogrid_Full/BESS Controller/DABCtrl2/Filter ICs/Internal IC - Differentiator ==
  D0 : Inport  SampleTime=SampleTime
  Ground : Ground  DisableCoverage=on
  Signal Specification : SignalSpecification  DisableCoverage=on  OutDataTypeStr=boolean  SampleTime=SampleTime
  Signal Specification1 : SignalSpecification  DisableCoverage=on  OutDataTypeStr=boolean  SampleTime=SampleTime
  Terminator : Terminator
  Out1 : Outport  SampleTime=SampleTime
  wires:
  D0/1 -> Signal Specification/1
  Signal Specification/1 -> Terminator/1
  Ground/1 -> Signal Specification1/1
  Signal Specification1/1 -> Out1/1

== system LunarMicrogrid_Full/BESS Controller/DABCtrl2/Filter ICs/Internal IC - Filter ==
  D0 : Inport  SampleTime=SampleTime
  Ground : Ground  DisableCoverage=on
  Signal Specification : SignalSpecification  DisableCoverage=on  OutDataTypeStr=boolean  SampleTime=SampleTime
  Signal Specification1 : SignalSpecification  DisableCoverage=on  OutDataTypeStr=boolean  SampleTime=SampleTime
  Terminator : Terminator
  Out1 : Outport  SampleTime=SampleTime
  wires:
  D0/1 -> Signal Specification/1
  Signal Specification/1 -> Terminator/1
  Ground/1 -> Signal Specification1/1
  Signal Specification1/1 -> Out1/1

== system LunarMicrogrid_Full/BESS Controller/DABCtrl2/I Gain/Disabled ==
  I Gain : Inport  SampleTime=SampleTime
  Signal Specification : SignalSpecification  DisableCoverage=on  OutDataTypeStr=boolean  SampleTime=SampleTime
  Terminator : Terminator
  wires:
  Signal Specification/1 -> Terminator/1
  I Gain/1 -> Signal Specification/1

== system LunarMicrogrid_Full/BESS Controller/DABCtrl2/I Gain/External Parameters ==
  err : Inport  SampleTime=SampleTime
  I Gain : Inport  Port=2  SampleTime=SampleTime
  IProd Out : Product  OutMin=IOutMin  OutMax=IOutMax  RndMeth=Simplest  SampleTime=SampleTime  OutDataTypeStr=Inherit: Same as first input
  Out1 : Outport  SampleTime=SampleTime
  wires:
  err/1 -> IProd Out/1
  I Gain/1 -> IProd Out/2
  IProd Out/1 -> Out1/1

== system LunarMicrogrid_Full/BESS Controller/DABCtrl2/I Gain/Internal Parameters ==
  err : Inport  SampleTime=SampleTime
  I Gain : Inport  Port=2  SampleTime=SampleTime
  Integral Gain : Gain  DisableCoverage=on  Gain=I  ParamMin=IParamMin  ParamMax=IParamMax  OutMin=IOutMin  OutMax=IOutMax  RndMeth=Simplest  OutDataTypeStr=Inherit: Same as input
  Signal Specification : SignalSpecification  DisableCoverage=on  OutDataTypeStr=boolean  SampleTime=SampleTime
  Terminator : Terminator
  Out1 : Outport  SampleTime=SampleTime
  wires:
  err/1 -> Integral Gain/1
  Integral Gain/1 -> Out1/1
  Signal Specification/1 -> Terminator/1
  I Gain/1 -> Signal Specification/1

== system LunarMicrogrid_Full/BESS Controller/DABCtrl2/Ideal P Gain/External Parameters ==
  In1 : Inport  SampleTime=SampleTime
  P Gain : Inport  Port=2  SampleTime=SampleTime
  PProd Out : Product  RndMeth=Simplest  SampleTime=SampleTime  OutDataTypeStr=Inherit: Same as first input
  Out1 : Outport  SampleTime=SampleTime
  wires:
  In1/1 -> PProd Out/1
  P Gain/1 -> PProd Out/2
  PProd Out/1 -> Out1/1

== system LunarMicrogrid_Full/BESS Controller/DABCtrl2/Ideal P Gain/Internal Parameters ==
  In1 : Inport  SampleTime=SampleTime
  P Gain : Inport  Port=2  SampleTime=SampleTime
  Proportional Gain : Gain  Gain=P  ParamMin=PParamMin  ParamMax=PParamMax  OutMin=POutMin  OutMax=POutMax  RndMeth=Simplest  OutDataTypeStr=Inherit: Same as input
  Signal Specification1 : SignalSpecification  DisableCoverage=on  OutDataTypeStr=boolean  SampleTime=SampleTime
  Terminator1 : Terminator
  Out1 : Outport  SampleTime=SampleTime
  wires:
  In1/1 -> Proportional Gain/1
  Proportional Gain/1 -> Out1/1
  P Gain/1 -> Signal Specification1/1
  Signal Specification1/1 -> Terminator1/1

== system LunarMicrogrid_Full/BESS Controller/DABCtrl2/Ideal P Gain/Passthrough ==
  In1 : Inport  SampleTime=SampleTime
  P Gain : Inport  Port=2  SampleTime=SampleTime
  Terminator1 : Terminator
  Out1 : Outport  SampleTime=SampleTime
  wires:
  In1/1 -> Out1/1
  P Gain/1 -> Terminator1/1

== system LunarMicrogrid_Full/BESS Controller/DABCtrl2/Ideal P Gain Fdbk/Disabled ==
  In1 : Inport  SampleTime=SampleTime
  P Gain : Inport  Port=2  SampleTime=SampleTime
  Signal Specification1 : SignalSpecification  DisableCoverage=on  OutDataTypeStr=boolean  SampleTime=SampleTime
  Terminator1 : Terminator
  Terminator2 : Terminator
  wires:
  P Gain/1 -> Terminator1/1
  In1/1 -> Signal Specification1/1
  Signal Specification1/1 -> Terminator2/1

== system LunarMicrogrid_Full/BESS Controller/DABCtrl2/Ideal P Gain Fdbk/External Parameters ==
  In1 : Inport  SampleTime=SampleTime
  P Gain : Inport  Port=2  SampleTime=SampleTime
  PProd Out : Product  RndMeth=Simplest  SampleTime=SampleTime  OutDataTypeStr=Inherit: Same as first input
  Out1 : Outport  SampleTime=SampleTime
  wires:
  PProd Out/1 -> Out1/1
  P Gain/1 -> PProd Out/2
  In1/1 -> PProd Out/1

== system LunarMicrogrid_Full/BESS Controller/DABCtrl2/Ideal P Gain Fdbk/Internal Parameters ==
  In1 : Inport  SampleTime=SampleTime
  P Gain : Inport  Port=2  SampleTime=SampleTime
  Proportional Gain : Gain  Gain=P  ParamMin=PParamMin  ParamMax=PParamMax  OutMin=POutMin  OutMax=POutMax  RndMeth=Simplest  OutDataTypeStr=Inherit: Same as input
  Signal Specification1 : SignalSpecification  DisableCoverage=on  OutDataTypeStr=boolean  SampleTime=SampleTime
  Terminator1 : Terminator
  Out1 : Outport  SampleTime=SampleTime
  wires:
  Proportional Gain/1 -> Out1/1
  In1/1 -> Proportional Gain/1
  Signal Specification1/1 -> Terminator1/1
  P Gain/1 -> Signal Specification1/1

== system LunarMicrogrid_Full/BESS Controller/DABCtrl2/Ideal P Gain Fdbk/Passthrough ==
  In1 : Inport  SampleTime=SampleTime
  P Gain : Inport  Port=2  SampleTime=SampleTime
  Terminator1 : Terminator
  Out1 : Outport  SampleTime=SampleTime
  wires:
  In1/1 -> Out1/1
  P Gain/1 -> Terminator1/1

== system LunarMicrogrid_Full/BESS Controller/DABCtrl2/Integrator/Continuous ==
  U : Inport  SampleTime=SampleTime
  Reset : Inport  Port=2  SampleTime=SampleTime
  I0in : Inport  Port=3  SampleTime=SampleTime
  Ground : Ground  DisableCoverage=on
  Integrator : Integrator
  Signal Specification1 : SignalSpecification  DisableCoverage=on  OutDataTypeStr=boolean  SampleTime=SampleTime
  Terminator : Terminator
  Terminator1 : Terminator
  state : Outport  SampleTime=SampleTime
  out : Outport  Port=2  SampleTime=SampleTime
  wires:
  U/1 -> Integrator/1
  I0in/1 -> Terminator/1
  Integrator/1 -> out/1
  Ground/1 -> Signal Specification1/1
  Signal Specification1/1 -> state/1
  Reset/1 -> Terminator1/1

== system LunarMicrogrid_Full/BESS Controller/DABCtrl2/Integrator/Disabled ==
  U : Inport  SampleTime=SampleTime
  Reset : Inport  Port=2  SampleTime=SampleTime
  I0in : Inport  Port=3  SampleTime=SampleTime
  Ground : Ground  DisableCoverage=on
  Signal Specification1 : SignalSpecification  DisableCoverage=on  OutDataTypeStr=boolean  SampleTime=SampleTime
  Signal Specification2 : SignalSpecification  DisableCoverage=on  OutDataTypeStr=boolean  SampleTime=SampleTime
  Signal Specification4 : SignalSpecification  DisableCoverage=on  OutDataTypeStr=boolean  SampleTime=SampleTime
  Terminator1 : Terminator
  Terminator2 : Terminator
  Terminator3 : Terminator
  out : Outport  SampleTime=SampleTime
  wires:
  Reset/1 -> Terminator2/1
  Signal Specification4/1 -> Terminator1/1
  I0in/1 -> Signal Specification4/1
  U/1 -> Signal Specification1/1
  Signal Specification1/1 -> Terminator3/1
  Ground/1 -> Signal Specification2/1
  Signal Specification2/1 -> out/1
